simulink model "SMDFR_rom_MCDET_v2_2022b"  (R2022b)
settings: Solver=ode1be  StartTime=0.0  StopTime=1500  FixedStep=0.5  RelTol=1e-3
model workspace: external: MATLAB File simulation_core_dualfluid_FI3_sim_rom_extract_MCDET_v2.m (data not in the file)
values from neighbouring files (symbols this model uses):
  A_fw = [13.6 9 9 9 9 9 9 9 9 9 9 13.6]    [SA_DualFluid.mat]
  A_wc = [10.9 10.3 10.3 10.3 10.3 10.3 10.3 10.3 10.3 10.3 10.3 10.9]    [SA_DualFluid.mat]
  h_fw = [6546 4305.1 4305.1 4305.1 4305.1 4305.1 4305.1 4305.1 4305.1 4305.1 4305.1 7629.5]    [SA_DualFluid.mat]
  h_wc = [27405.4 13833.4 13833.4 13833.4 13833.4 13833.4 13833.4 13833.4 13833.4 13833.4 13833.4 32177.3]    [SA_DualFluid.mat]
  Ncomps = 5    [LJ_test_sampled_vel_ACS_2_loop_1180.mat]
undefined symbols (not defined in the file or in its folder): alfa_c, alfa_f, beta, beta_i, C_i0, c_pc, c_pf, c_pw, Ce_i0, complementary_branch_flag, DiscIntNeverNeededParam, failed_states, fault_time, initial_branch_state, initial_state, L, Lambda, lambda_c, lambda_e, lambda_i, M_c, M_f, M_w, mat_states_index, mat_trans, mdot_c, mdot_c_drift, mdot_f, N_0, Nstates, P_0, parent_last_time, Pi_0, rho_0, rhoex_value, Tbar_c0, Tbar_f0, Tc_0, Tf_0, Tin_f0, Tw_0, vel_ACS
libraries: dspsrcs4 x1
settings Model: Creator=leona  LastModifiedBy=leona
settings DataIOCC: LoadExternalInput=on
settings OptimizationCC: ReuseModelBlockBuffer=on

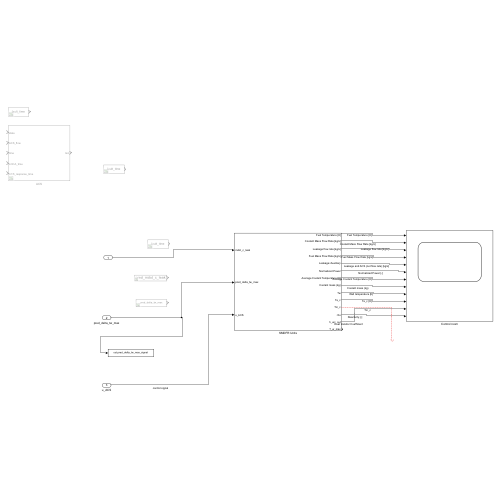
[thumbnail: Simulink's stored preview of the top-level diagram]
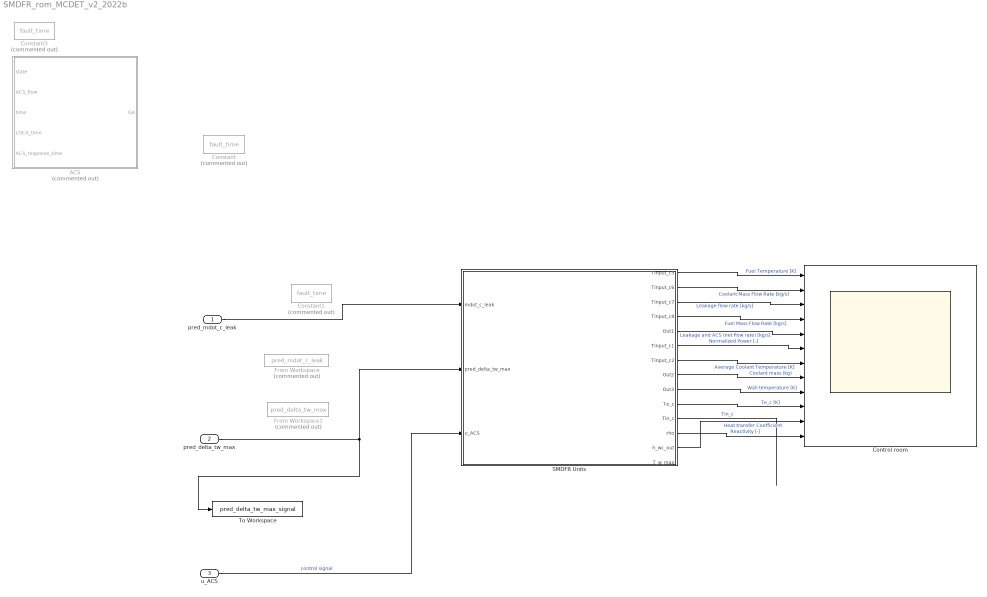
== system SMDFR_rom_MCDET_v2_2022b ==
  pred_mdot_c_leak : Inport
  pred_delta_tw_max : Inport  Port=2
  u_ACS : Inport  Port=3
  ACS : Subsystem  Commented=on
  Constant : Constant  Commented=on  Value=fault_time
  Constant1 : Constant  Commented=on  Value=fault_time
  Constant3 : Constant  Commented=on  Value=fault_time
  Control room : Scope  NumInputPorts=12
  From Workspace : FromWorkspace  Commented=on  VariableName=pred_mdot_c_leak  SampleTime=0.5  Interpolate=off  OutputAfterFinalValue=Holding final value
  From Workspace1 : FromWorkspace  Commented=on  VariableName=pred_delta_tw_max  SampleTime=0.5  OutputAfterFinalValue=Holding final value
  SMDFR Units : Subsystem
  To Workspace : ToWorkspace  VariableName=pred_delta_tw_max_signal  SaveFormat=Timeseries  SampleTime=-1
  wires:
  SMDFR Units/1(Tinput_c5) -> Control room/1  "Fuel Temperature [K]"
  SMDFR Units/2(Tinput_c6) -> Control room/2  "Coolant Mass Flow Rate [kg/s]"
  SMDFR Units/3(Tinput_c7) -> Control room/3  "Leakage flow rate [kg/s]"
  SMDFR Units/4(Tinput_c8) -> Control room/4  "Fuel Mass Flow Rate [kg/s]"
  SMDFR Units/5(Out1) -> Control room/5  "Leakage and ACS (net flow rate) [kg/s]"
  SMDFR Units/6(Tinput_c1) -> Control room/6  "Normalized Power [-]"
  SMDFR Units/7(Tinput_c2) -> Control room/7  "Average Coolant Temperature [K]"
  SMDFR Units/8(Out2) -> Control room/8  "Coolant mass (kg)"
  SMDFR Units/9(Out3) -> Control room/9  "Wall temperature [K]"
  SMDFR Units/10(Te_c) -> Control room/10  "Te_c [K]"
  SMDFR Units/11(Tin_c) -> ?  "Tin_c"
  SMDFR Units/12(rho) -> Control room/12  "Reactivity [-]"
  SMDFR Units/13(h_wc_out) -> Control room/11  "Heat transfer Coefficient"
  pred_delta_tw_max/1 -> To Workspace/1, SMDFR Units/2(pred_delta_tw_max)
  pred_mdot_c_leak/1 -> SMDFR Units/1(mdot_c_leak)
  u_ACS/1 -> SMDFR Units/3(u_ACS)  "control signal"

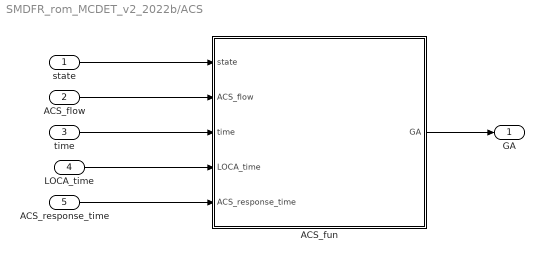
== system SMDFR_rom_MCDET_v2_2022b/ACS ==
  state : Inport
  ACS_flow : Inport  Port=2
  time : Inport  Port=3
  LOCA_time : Inport  Port=4
  ACS_response_time : Inport  Port=5
  ACS_fun : MATLAB Function  TreatAsAtomicUnit=on
  GA : Outport
  wires:
  ACS_flow/1 -> ACS_fun/2(ACS_flow)
  state/1 -> ACS_fun/1(state)
  ACS_fun/1(GA) -> GA/1
  time/1 -> ACS_fun/3(time)
  LOCA_time/1 -> ACS_fun/4(LOCA_time)
  ACS_response_time/1 -> ACS_fun/5(ACS_response_time)

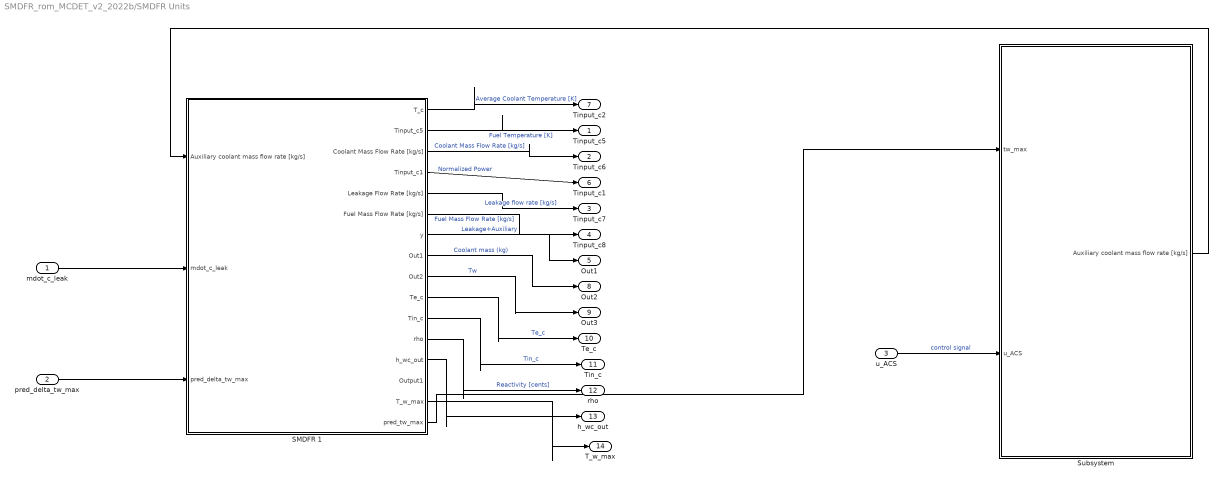
== system SMDFR_rom_MCDET_v2_2022b/SMDFR Units ==
  mdot_c_leak : Inport
  pred_delta_tw_max : Inport  Port=2
  u_ACS : Inport  Port=3
  SMDFR 1 : Subsystem
  Subsystem : Subsystem
  Tinput_c5 : Outport
  Tinput_c6 : Outport  Port=2
  Tinput_c7 : Outport  Port=3
  Tinput_c8 : Outport  Port=4
  Out1 : Outport  Port=5
  Tinput_c1 : Outport  Port=6
  Tinput_c2 : Outport  Port=7
  Out2 : Outport  Port=8
  Out3 : Outport  Port=9
  Te_c : Outport  Port=10
  Tin_c : Outport  Port=11
  rho : Outport  Port=12
  h_wc_out : Outport  Port=13
  T_w_max : Outport  Port=14
  wires:
  SMDFR 1/10(Te_c) -> Te_c/1  "Te_c"
  SMDFR 1/8(Out1) -> Out2/1  "Coolant mass (kg)"
  SMDFR 1/12(rho) -> rho/1  "Reactivity [cents]"
  SMDFR 1/9(Out2) -> Out3/1  "Tw"
  SMDFR 1/1(T_c) -> Tinput_c2/1  "Average Coolant Temperature [K]"
  SMDFR 1/3(Coolant Mass Flow Rate [kg/s]) -> Tinput_c6/1  "Coolant Mass Flow Rate [kg/s]"
  SMDFR 1/11(Tin_c) -> Tin_c/1  "Tin_c"
  SMDFR 1/6(Fuel Mass Flow Rate [kg/s]) -> Tinput_c8/1  "Fuel Mass Flow Rate [kg/s]"
  SMDFR 1/4(Tinput_c1) -> Tinput_c1/1  "Normalized Power"
  SMDFR 1/7(y) -> Out1/1  "Leakage+Auxiliary"
  SMDFR 1/2(Tinput_c5) -> Tinput_c5/1  "Fuel Temperature [K]"
  SMDFR 1/5(Leakage Flow Rate [kg/s]) -> Tinput_c7/1  "Leakage flow rate [kg/s]"
  Subsystem/1(Auxiliary coolant mass flow rate [kg/s]) -> SMDFR 1/1(Auxiliary coolant mass flow rate [kg/s])
  SMDFR 1/13(h_wc_out) -> h_wc_out/1
  SMDFR 1/15(T_w_max) -> T_w_max/1
  SMDFR 1/16(pred_tw_max) -> Subsystem/1(tw_max)
  mdot_c_leak/1 -> SMDFR 1/2(mdot_c_leak)
  pred_delta_tw_max/1 -> SMDFR 1/3(pred_delta_tw_max)
  u_ACS/1 -> Subsystem/2(u_ACS)  "control signal"

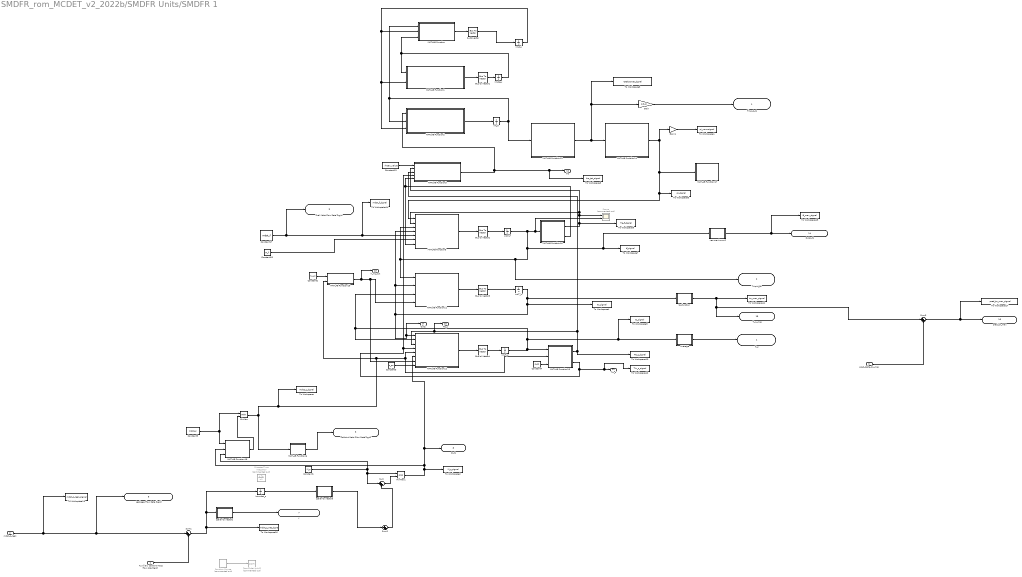
== system SMDFR_rom_MCDET_v2_2022b/SMDFR Units/SMDFR 1 ==
  Auxiliary coolant mass flow rate [kg/s] : Inport
  mdot_c_leak : Inport  Port=2
  pred_delta_tw_max : Inport  Port=3
  Average : MATLAB Function  TreatAsAtomicUnit=on
  Bus to Vector{1..4} (4 alike) : BusToVector
  Constant1 : Constant  Value=M_c
  Constant13 : Constant  Value=rhoex_value  SampleTime=-1
  Constant17 : Constant  Value=mdot_f  SampleTime=-1
  Constant2 : Constant  Value=h_wc
  Constant20 : Constant  Value=M_f  SampleTime=-1
  Constant3 : Constant  Value=c_pc
  Constant4 : Constant  Value=c_pc
  Constant9 : Constant  Value=mdot_c  SampleTime=-1
  Discrete-Time Integrator : DiscreteIntegrator  Commented=on  SampleTime=0.5  ICPrevOutput=DiscIntNeverNeededParam  ICPrevScaledInput=DiscIntNeverNeededParam
  Gain : Gain  Gain=1/P_0
  Gain1 : Gain  Gain=1/P_0
  Int-C_i : Integrator  InitialCondition=C_i0
  Int-Ce_i : Integrator  InitialCondition=Ce_i0
  Int-T_c : Integrator  InitialCondition=Tc_0
  Int-T_f : Integrator  InitialCondition=Tf_0
  Int-T_w : Integrator  InitialCondition=Tw_0
  Int-mdot_c : Integrator
  Int_N : Integrator  InitialCondition=N_0
  MATLAB Function : MATLAB Function  TreatAsAtomicUnit=on
  MATLAB Function1 : MATLAB Function  TreatAsAtomicUnit=on
  MATLAB Function11 : MATLAB Function  TreatAsAtomicUnit=on
  MATLAB Function12 : MATLAB Function  TreatAsAtomicUnit=on
  MATLAB Function13 : MATLAB Function  TreatAsAtomicUnit=on
  MATLAB Function14 : MATLAB Function  TreatAsAtomicUnit=on
  MATLAB Function15 : MATLAB Function  TreatAsAtomicUnit=on
  MATLAB Function16 : MATLAB Function  TreatAsAtomicUnit=on
  MATLAB Function17 : MATLAB Function  TreatAsAtomicUnit=on
  MATLAB Function18 : MATLAB Function  TreatAsAtomicUnit=on
  MATLAB Function19 : MATLAB Function  TreatAsAtomicUnit=on
  MATLAB Function2 : MATLAB Function  TreatAsAtomicUnit=on
  MATLAB Function3 : MATLAB Function  TreatAsAtomicUnit=on
  MATLAB Function5 : MATLAB Function  TreatAsAtomicUnit=on
  MATLAB Function6 : MATLAB Function  TreatAsAtomicUnit=on
  MinMax : MinMax  Inputs=2
  MinMax1 : MinMax  Inputs=2
  Random Source : dspsrcs4/Random Source  Commented=on  SrcType=Gaussian  NormMethod=Ziggurat  CltLength=12  MinVal=0  MaxVal=1  MeanVal=0  VarVal=0.05*mdot_c_drift  RepMode=Not repeatable  rawSeed=1  IsInherit=off  SampMode=Discrete  SampTime=-1  SampFrame=1  DataType=Double  OutComplex=Real  OutputFrames=off
  Scope : Scope  Commented=on  NumInputPorts=2
  Sum{,1..3} (4 alike) : Sum  Inputs=|++
  To Workspace : ToWorkspace  VariableName=mdot_c_signal  SaveFormat=Timeseries  SampleTime=-1
  To Workspace1 : ToWorkspace  VariableName=pi_normsignal  SaveFormat=Timeseries  SampleTime=-1
  To Workspace10 : ToWorkspace  VariableName=Te_c_signal  SaveFormat=Timeseries  SampleTime=-1
  To Workspace11 : ToWorkspace  VariableName=tw_max_signal  SaveFormat=Timeseries  SampleTime=-1
  To Workspace12 : ToWorkspace  VariableName=Tin_c_signal  SaveFormat=Timeseries  SampleTime=-1
  To Workspace13 : ToWorkspace  VariableName=mdot_c_leak_signal  SaveFormat=Timeseries  SampleTime=-1
  To Workspace14 : ToWorkspace  VariableName=mdot_f_signal  SaveFormat=Timeseries  SampleTime=-1
  To Workspace15 : ToWorkspace  VariableName=tf_max_signal  SaveFormat=Timeseries  SampleTime=-1
  To Workspace16 : ToWorkspace  VariableName=mdot_c_net_signal  SaveFormat=Timeseries  SampleTime=-1
  To Workspace17 : ToWorkspace  VariableName=pred_tw_max_signal  SaveFormat=Timeseries  SampleTime=-1
  To Workspace2 : ToWorkspace  VariableName=M_c_signal  SaveFormat=Timeseries  SampleTime=-1
  To Workspace3 : ToWorkspace  VariableName=totalpower_signal  SaveFormat=Timeseries  SampleTime=-1
  To Workspace4 : ToWorkspace  VariableName=tw_signal  SaveFormat=Timeseries  SampleTime=-1
  To Workspace5 : ToWorkspace  VariableName=tc_signal  SaveFormat=Timeseries  SampleTime=-1
  To Workspace6 : ToWorkspace  VariableName=pi_signal  SaveFormat=Timeseries  SampleTime=-1
  To Workspace7 : ToWorkspace  VariableName=tf_signal  SaveFormat=Timeseries  SampleTime=-1
  To Workspace8 : ToWorkspace  VariableName=rho_tot_signal  SaveFormat=Timeseries  SampleTime=-1
  To Workspace9 : ToWorkspace  VariableName=Te_f_signal  SaveFormat=Timeseries  SampleTime=-1
  Zero-Order Hold2 : ZeroOrderHold  Commented=on  SampleTime=-1
  bustovector : BusToVector
  scalar to vector2 : MATLAB Function  TreatAsAtomicUnit=on
  scalar to vector3 : MATLAB Function  TreatAsAtomicUnit=on
  tp_function : MATLAB Function  TreatAsAtomicUnit=on
  vec maximum2 : MATLAB Function  TreatAsAtomicUnit=on
  T_c : Outport
  Tinput_c5 : Outport  Port=2
  Coolant Mass Flow Rate [kg/s] : Outport  Port=3
  Tinput_c1 : Outport  Port=4
  Leakage Flow Rate [kg/s] : Outport  Port=5
  Fuel Mass Flow Rate [kg/s] : Outport  Port=6
  y : Outport  Port=7
  Out1 : Outport  Port=8
  Out2 : Outport  Port=9
  Te_c : Outport  Port=10
  Tin_c : Outport  Port=11
  rho : Outport  Port=12
  h_wc_out : Outport  Port=13
  Output1 : Outport  Port=14
  T_w_max : Outport  Port=15
  pred_tw_max : Outport  Port=16
  wires:
  Constant20/1 -> MATLAB Function5/6(M_f)
  bustovector/1 -> Int-C_i/1
  Constant13/1 -> MATLAB Function3/1(rho_ext)
  Int-T_w/1 -> To Workspace4/1, Out2/1, MATLAB Function12/1(T_w), MATLAB Function5/4(T_w), MATLAB Function11/2(T_w), tp_function/1(T_w)  "Tw"
  MinMax/1 -> To Workspace/1, MATLAB Function19/2(mdot_c), MATLAB Function15/2(mdot_c), MATLAB Function12/5(mdot_c), MATLAB Function6/1(u)  "Coolant mass flow rate (kg/s)"
  scalar to vector2/1(y) -> y/1  "Auxiliary+leakage"
  MATLAB Function15/1(Te_c) -> To Workspace10/1, MATLAB Function3/3(Te_c), MATLAB Function12/3(Te_c), Te_c/1  "Te_c"
  MATLAB Function16/1(Te_f) -> To Workspace9/1, Scope/1, MATLAB Function3/2(Te_f), MATLAB Function5/2(Te_f)
  Constant17/1 -> Fuel Mass Flow Rate [kg/s]/1, To Workspace14/1, MATLAB Function5/5(mdot_f)  "Fuel mass flow rate (kg/s)"
  Bus to Vector4/1 -> Int-T_c/1
  MATLAB Function11/1(dT_wdt) -> Bus to Vector3/1
  MATLAB Function/1(dC_idt) -> bustovector/1
  MATLAB Function3/1(rho) -> MATLAB Function2/1(rho), To Workspace8/1, rho/1  "Total Reactivity (cents)"
  Constant9/1 -> MATLAB Function18/1(mdot_c), MinMax/1
  Int-Ce_i/1 -> MATLAB Function/3(Ce_i), MATLAB Function1/1(Ce_i)
  MATLAB Function12/1(dT_cdt) -> Bus to Vector4/1
  MATLAB Function13/1(P) -> To Workspace3/1, Gain/1, MATLAB Function14/1(P)
  MATLAB Function14/1(Pi) -> To Workspace6/1, MATLAB Function5/1(Pi), MATLAB Function17/1(Pi), Gain1/1
  MATLAB Function5/1(dT_fdt) -> Bus to Vector2/1
  Bus to Vector2/1 -> Int-T_f/1
  Bus to Vector1/1 -> Int-Ce_i/1
  MATLAB Function1/1(dCei_dt) -> Bus to Vector1/1
  Int-C_i/1 -> MATLAB Function2/3(C_i), MATLAB Function1/2(C_i), MATLAB Function/2(C_i)
  MATLAB Function2/1(dN_dt) -> Int_N/1
  Int_N/1 -> MATLAB Function13/1(N), MATLAB Function/1(N), MATLAB Function2/2(N)
  Bus to Vector3/1 -> Int-T_w/1
  Average/1(y) -> T_c/1  "Average Coolant Temperature [K]"
  Int-T_c/1 -> MATLAB Function12/2(T_c), MATLAB Function11/3(T_c), To Workspace5/1, Average/1(u), MATLAB Function15/1(T_c)  "Coolant Temperature [K]"
  MATLAB Function6/1(y) -> Coolant Mass Flow Rate [kg/s]/1
  Auxiliary coolant mass flow rate [kg/s]/1 -> Sum1/2  "Auxiliary coolant mass flow rate [kg/s]"
  MATLAB Function18/1(y) -> MinMax/2  "Coolant mass flow rate (kg/s)"
  scalar to vector3/1(y) -> Sum2/1  "Coolant mass per node (kg)"
  Constant1/1 -> Sum/1, MinMax1/1, MATLAB Function18/3(M_total)
  MATLAB Function15/2(Tin_c) -> MATLAB Function3/4(Tin_c), MATLAB Function12/4(Tinput_c), To Workspace12/1, Tin_c/1  "Tin_c"
  MinMax1/1 -> To Workspace2/1, MATLAB Function12/6(M_c), Out1/1, MATLAB Function18/2(M_actual)  "Coolant mass (kg)"
  Constant2/1 -> MATLAB Function19/1(h_wc)
  MATLAB Function19/1(h_wc_out) -> h_wc_out/1, MATLAB Function12/7(h_wc), MATLAB Function11/4(h_wc)
  Sum/1 -> MinMax1/2  "Coolant mass (kg)"
  Random Source/1 -> Zero-Order Hold2/1
  Gain/1 -> Tinput_c1/1  "Normalized Power"
  Gain1/1 -> To Workspace1/1
  MATLAB Function16/2(Tin_f) -> MATLAB Function3/5(Tin_f), MATLAB Function5/7(Tin_f)
  Int-mdot_c/1 -> scalar to vector3/1(u)  "Coolant mass per node (kg)"
  Int-T_f/1 -> vec maximum2/1(T_f), To Workspace7/1, Tinput_c5/1, MATLAB Function11/1(T_f), MATLAB Function5/3(T_f), Scope/2, MATLAB Function16/1(T_f)  "Fuel temperature profile (K)"
  vec maximum2/1(y) -> To Workspace15/1, Output1/1  "T_f_max"
  Sum2/1 -> Sum/2
  Constant3/1 -> MATLAB Function12/8(c_pc)
  Constant4/1 -> MATLAB Function15/3(c_pc)
  Sum1/1 -> Int-mdot_c/1, scalar to vector2/1(u), To Workspace16/1
  mdot_c_leak/1 -> Sum1/1, Leakage Flow Rate [kg/s]/1, To Workspace13/1
  Sum3/1 -> To Workspace17/1, pred_tw_max/1
  pred_delta_tw_max/1 -> Sum3/2
  tp_function/1(T_p) -> Sum3/1, T_w_max/1, To Workspace11/1

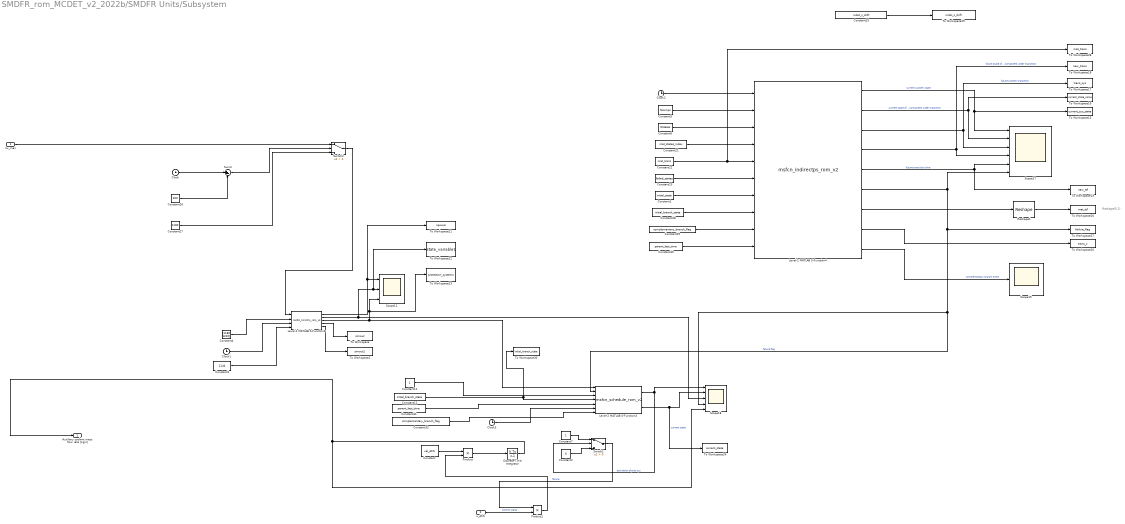
== system SMDFR_rom_MCDET_v2_2022b/SMDFR Units/Subsystem ==
  note: Reshape(5,2)
  tw_max : Inport
  u_ACS : Inport  Port=2
  Clock{,1..3} (4 alike) : Clock
  Constant : Constant  Value=vel_ACS
  Constant1 : Constant  Value=initial_state
  Constant11 : Constant  Value=initial_branch_state
  Constant12 : Constant
  Constant2 : Constant  Value=0
  Constant21 : Constant  Value=mat_states_index
  Constant22 : Constant  Value=mat_trans
  Constant23 : Constant  Value=failed_states
  Constant25 : Constant  Value=mdot_c_drift
  Constant26 : Constant  Value=200
  Constant27 : Constant  Value=1100
  Constant28 : Constant  Value=initial_branch_state
  Constant29 : Constant  Value=complementary_branch_flag
  Constant3 : Constant  Value=1144
  Constant30 : Constant  Value=parent_last_time
  Constant31 : Constant  Value=parent_last_time
  Constant32 : Constant  Value=complementary_branch_flag
  Constant4 : Constant  Value=[1180 1220]
  Constant5 : Constant  Value=Ncomps
  Constant6 : Constant  Value=Nstates
  Constant7 : Constant
  Discrete-Time Integrator : DiscreteIntegrator  SampleTime=-1  ICPrevOutput=DiscIntNeverNeededParam  ICPrevScaledInput=DiscIntNeverNeededParam
  Level-2 MATLAB S-Function2 : M-S-Function  FunctionName=msfcn_limintm_rom_v2
  Level-2 MATLAB S-Function3 : M-S-Function  FunctionName=msfcn_schedule_rom_v2
  Level-2 MATLAB S-Function4 : M-S-Function  FunctionName=msfcn_indirectps_rom_v2
  Product : Product
  Product1 : Product
  Reshape1 : Reshape  OutputDimensionality=Customize  OutputDimensions=[5,2]
  Scope11 : Scope  NumInputPorts=3
  Scope15 : Scope
  Scope17 : Scope  NumInputPorts=6
  Scope18 : Scope  NumInputPorts=5
  Sum3 : Sum  Inputs=|+-
  Switch1 : Switch  Criteria=u2 > Threshold  SaturateOnIntegerOverflow=off  InputSameDT=off
  Switch2 : Switch  Criteria=u2 > Threshold  SaturateOnIntegerOverflow=off  InputSameDT=off
  To Workspace : ToWorkspace  VariableName=simout  SaveFormat=Timeseries  SampleTime=-1
  To Workspace1 : ToWorkspace  VariableName=simout1  SaveFormat=Timeseries  SampleTime=-1
  To Workspace15 : ToWorkspace  VariableName=current_sys_state  SaveFormat=Timeseries  SampleTime=-1
  To Workspace16 : ToWorkspace  VariableName=current_state_comp  SaveFormat=Timeseries  SampleTime=-1
  To Workspace17 : ToWorkspace  VariableName=trans_sys  SaveFormat=Timeseries  SampleTime=-1
  To Workspace18 : ToWorkspace  VariableName=new_trans  SaveFormat=Timeseries  SampleTime=-1
  To Workspace19 : ToWorkspace  VariableName=new_ttf  SaveFormat=Timeseries  SampleTime=-1
  To Workspace20 : ToWorkspace  VariableName=trans_c  SaveFormat=Timeseries  SampleTime=-1
  To Workspace21 : ToWorkspace  VariableName=npower  SaveFormat=Timeseries  SampleTime=-1
  To Workspace22 : ToWorkspace  VariableName=state_variable1  SaveFormat=Timeseries  SampleTime=-1
  To Workspace23 : ToWorkspace  VariableName=protection_systems  SaveFormat=Timeseries  SampleTime=-1
  To Workspace24 : ToWorkspace  VariableName=current_state  SaveFormat=Timeseries  SampleTime=-1
  To Workspace26 : ToWorkspace  VariableName=mat_ttf  SaveFormat=Timeseries  SampleTime=-1
  To Workspace27 : ToWorkspace  VariableName=failure_flag  SaveFormat=Timeseries  SampleTime=-1
  To Workspace28 : ToWorkspace  VariableName=mat_trans  SaveFormat=Timeseries  SampleTime=-1
  To Workspace29 : ToWorkspace  VariableName=mdot_c_drift  SaveFormat=Timeseries  SampleTime=-1
  To Workspace30 : ToWorkspace  VariableName=initial_branch_state  SaveFormat=Timeseries  SampleTime=-1
  Auxiliary coolant mass flow rate [kg/s] : Outport
  wires:
  Level-2 MATLAB S-Function4/6 -> Level-2 MATLAB S-Function3/2, Scope18/4, To Workspace27/1, Scope17/6  "failure flag"
  Constant6/1 -> Level-2 MATLAB S-Function4/3
  Level-2 MATLAB S-Function4/9 -> Scope15/1  "complementary branch event"
  Sum3/1 -> Switch2/2
  Level-2 MATLAB S-Function4/5 -> To Workspace19/1, Scope17/5  "future transition time"
  Constant23/1 -> Level-2 MATLAB S-Function4/6
  Constant28/1 -> Level-2 MATLAB S-Function4/8
  Clock2/1 -> Level-2 MATLAB S-Function4/1
  Level-2 MATLAB S-Function2/2 -> Scope18/3, To Workspace22/1, Scope11/2
  Constant22/1 -> To Workspace28/1, Level-2 MATLAB S-Function4/5
  Discrete-Time Integrator/1 -> Auxiliary coolant mass flow rate [kg/s]/1, Scope18/5
  Level-2 MATLAB S-Function3/2 -> To Workspace24/1, Scope18/2  "current state"
  Level-2 MATLAB S-Function4/1 -> Scope17/1, To Workspace15/1  "current system state"
  Level-2 MATLAB S-Function4/4 -> Scope17/4, To Workspace18/1  "future state of component under transition"
  Clock3/1 -> Level-2 MATLAB S-Function3/6
  Constant21/1 -> Level-2 MATLAB S-Function4/4
  Constant32/1 -> Level-2 MATLAB S-Function3/7
  Level-2 MATLAB S-Function2/3 -> To Workspace23/1, Scope11/3, Level-2 MATLAB S-Function3/1
  Constant11/1 -> To Workspace30/1, Level-2 MATLAB S-Function3/4
  Constant30/1 -> Level-2 MATLAB S-Function4/10
  Constant31/1 -> Level-2 MATLAB S-Function3/5
  Reshape1/1 -> To Workspace26/1
  Constant12/1 -> Level-2 MATLAB S-Function3/3
  Level-2 MATLAB S-Function4/3 -> Scope17/3, To Workspace17/1  "future system transition"
  Clock/1 -> Sum3/1
  Clock1/1 -> Level-2 MATLAB S-Function2/3
  Constant1/1 -> Level-2 MATLAB S-Function4/7
  Level-2 MATLAB S-Function4/2 -> Scope17/2, To Workspace16/1  "current state of component under transition"
  Constant3/1 -> Level-2 MATLAB S-Function2/4
  Constant4/1 -> Level-2 MATLAB S-Function2/2
  Level-2 MATLAB S-Function4/7 -> Reshape1/1
  Constant7/1 -> Switch1/1
  Constant2/1 -> Switch1/3
  Level-2 MATLAB S-Function2/1 -> To Workspace21/1, Scope11/1
  Switch2/1 -> Level-2 MATLAB S-Function2/1
  Constant27/1 -> Switch2/3
  Constant26/1 -> Sum3/2
  Constant29/1 -> Level-2 MATLAB S-Function4/9
  Level-2 MATLAB S-Function3/1 -> Switch1/2, Scope18/1  "activation of prot sys"
  Constant5/1 -> Level-2 MATLAB S-Function4/2
  Level-2 MATLAB S-Function4/8 -> To Workspace20/1
  Constant25/1 -> To Workspace29/1
  tw_max/1 -> Switch2/1
  Level-2 MATLAB S-Function2/4 -> To Workspace/1
  Level-2 MATLAB S-Function2/5 -> To Workspace1/1
  Switch1/1 -> Product1/1  "failure"
  Constant/1 -> Product/1
  Product/1 -> Discrete-Time Integrator/1
  u_ACS/1 -> Product1/2  "control signal"
  Product1/1 -> Product/2

== matlab function SMDFR_rom_MCDET_v2_2022b/SMDFR Units/SMDFR 1/tp_function ==
  data: T_w input size=1; T_p output
function T_p = fcn(T_w)

T_p = max(T_w);

== matlab function SMDFR_rom_MCDET_v2_2022b/SMDFR Units/SMDFR 1/MATLAB Function11 ==
  data: T_f input size=1; T_w input size=1; dT_wdt output size=1; T_c input size=1; A_wc parameter size=1; A_fw parameter size=1; M_w parameter size=1; c_pw parameter size=1; h_wc input size=1; h_fw parameter size=1
function dT_wdt = eqn9(T_f, T_w, T_c, A_wc, A_fw, M_w, c_pw, h_wc, h_fw)
%dT_wdt = 0;

dT_wdt = ( h_fw*A_fw*(T_f - T_w) - h_wc*A_wc*(T_w -T_c) ) / (M_w * c_pw);

== matlab function SMDFR_rom_MCDET_v2_2022b/SMDFR Units/SMDFR 1/MATLAB Function12 ==
  data: T_w input size=1; T_c input size=1; A_wc parameter size=1; dT_cdt output size=1; Te_c input size=1; Tinput_c input; mdot_c input size=1; M_c input size=1; h_wc input size=1; c_pc input size=1
function dT_cdt = eqn10(T_w, T_c, A_wc, Te_c, Tinput_c, mdot_c, M_c, h_wc, c_pc)
%!!!
dT_cdt = 0;
%Tinput_c=Tinput_c(1);

dT_cdt = ( mdot_c*c_pc*(Tinput_c - Te_c) + h_wc*A_wc*(T_w - T_c) ) / (M_c * c_pc);

== matlab function SMDFR_rom_MCDET_v2_2022b/SMDFR Units/SMDFR 1/MATLAB Function13 ==
  data: P output; N input; N_0 parameter; P_0 parameter
function P = eqn14(N, N_0, P_0)
%P = P_0;

P = (P_0/N_0) * N;

== matlab function SMDFR_rom_MCDET_v2_2022b/SMDFR Units/SMDFR 1/MATLAB Function14 ==
  data: Pi output size=1; P input; Pi_0 parameter size=1; P_0 parameter
function Pi = distr(P, Pi_0, P_0)
Pi = 0;
%Pi = P_0*Pi_0';

Pi = P*Pi_0;

== matlab function SMDFR_rom_MCDET_v2_2022b/SMDFR Units/SMDFR 1/MATLAB Function15 ==
  data: T_c input size=1; Te_c output size=1; Te_c0 parameter size=1; mdot_c input size=1; Tin_c output size=1; c_pc input size=1
function [Te_c, Tin_c]  = cons1(T_c, Te_c0, mdot_c, c_pc)
%Te_c = tc_last;
%!!!
Te_c = Te_c0;

Q0 = 8.2564e+07*0.578;
Q = Q0*mdot_c(1)/(5550/2)-(5500-mdot_c);
Tin_c = Te_c-Q/(mean(mdot_c)*c_pc);

Te_c = 2*T_c - Tin_c;

== matlab function SMDFR_rom_MCDET_v2_2022b/SMDFR Units/SMDFR 1/MATLAB Function16 ==
  data: T_f input size=1; Te_f output size=1; Te_f0 parameter size=1; Tin_f output size=1
 function [Te_f, Tin_f] = cons1(T_f,Te_f0)
%Te_f = tf_last;
%Te_f = zeros(3,1);
%Te_f(2) = Te_f0(2);
%Te_f(3) = Te_f0(3);
%!!!
Te_f = Te_f0;
Tin_f = Te_f;
%Te_f(1) = Te_f0(1);

Te_f = 2*T_f - Tin_f;

== matlab function SMDFR_rom_MCDET_v2_2022b/SMDFR Units/SMDFR 1/MATLAB Function17 ==
  data: Pi input size=1; sum_P output
function sum_P = fcn(Pi)

sum_P = sum(Pi);

== matlab function SMDFR_rom_MCDET_v2_2022b/SMDFR Units/SMDFR 1/MATLAB Function18 ==
  data: mdot_c input; y output; M_actual input; M_total input
function y = fcn(mdot_c,M_actual,M_total)
y=0;

%y = mdot_c+Auxiliary_leakage*(time-LOCA_time);
y = mdot_c*M_actual/M_total;

== matlab function SMDFR_rom_MCDET_v2_2022b/SMDFR Units/SMDFR 1/vec maximum2 ==
  data: T_f input; y output
function y = fcn(T_f)

y = max(T_f);

== matlab function SMDFR_rom_MCDET_v2_2022b/SMDFR Units/SMDFR 1/MATLAB Function19 ==
  data: h_wc input; h_wc_out output; mdot_c input
function h_wc_out = fcn(h_wc,mdot_c)

h_wc_out=0;

h_wc_out=h_wc*(mdot_c/5550)^(0.8);

== matlab function SMDFR_rom_MCDET_v2_2022b/SMDFR Units/SMDFR 1/scalar to vector2 ==
  data: u input; y output
function y = fcn(u)
%!!!
y = 0;

y = u;

== matlab function SMDFR_rom_MCDET_v2_2022b/SMDFR Units/SMDFR 1/MATLAB Function6 ==
  data: u input; y output
function y = fcn(u)

y = mean(u);

== matlab function SMDFR_rom_MCDET_v2_2022b/SMDFR Units/SMDFR 1/MATLAB Function1 ==
  data: Ce_i input size=6,1; dCei_dt output size=6,1; C_i input size=6,1; lambda_i parameter size=1,6; lambda_e parameter; lambda_c parameter; L parameter
function dCei_dt = eqn3(Ce_i, C_i, lambda_i, lambda_e, lambda_c, L)
dCei_dt = zeros(6,1); %!!!

for i=1:L 
    dCei_dt(i) = -lambda_i(i)*Ce_i(i) - lambda_e*Ce_i(i) + lambda_c*C_i(i) ;
end

== matlab function SMDFR_rom_MCDET_v2_2022b/ACS/ACS_fun ==
  data: state input; GA output; ACS_flow input; time input; LOCA_time input; ACS_response_time input
function GA  = ACS(state,ACS_flow,time,LOCA_time,ACS_response_time)

if state && (time-LOCA_time) > ACS_response_time
    GA = ACS_flow;
else
    GA = 0;
end

== matlab function SMDFR_rom_MCDET_v2_2022b/SMDFR Units/SMDFR 1/MATLAB Function ==
  data: N input; dC_idt output size=6,1; C_i input size=6,1; Ce_i input size=6,1; Lambda parameter; lambda_i parameter size=1,6; lambda_c parameter; lambda_e parameter; beta_i parameter size=1,6
function dC_idt = eqn2(N, C_i, Ce_i, Lambda, lambda_i, lambda_c, lambda_e, beta_i)
dC_idt = zeros(6,1);

for i=1:6
    dC_idt(i) = beta_i(i)/Lambda * N - lambda_i(i)*C_i(i) - lambda_c*C_i(i) + lambda_e*Ce_i(i);
end

== matlab function SMDFR_rom_MCDET_v2_2022b/SMDFR Units/SMDFR 1/MATLAB Function2 ==
  data: rho input; dN_dt output; N input; C_i input size=6,1; lambda_i parameter size=1,6; beta parameter; Lambda parameter; L parameter
function dN_dt = eqn4(rho, N, C_i, lambda_i, beta, Lambda, L)
sum_i = 0;

for i=1:L 
    sum_i = sum_i + lambda_i(i)*C_i(i);
end

dN_dt = (rho - beta)*(N/Lambda) + sum_i;

== matlab function SMDFR_rom_MCDET_v2_2022b/SMDFR Units/SMDFR 1/MATLAB Function3 ==
  data: rho_ext input; rho output; rho_0 parameter; Te_f input; Te_c input; Tbar_f0 parameter; Tbar_c0 parameter; alfa_f parameter; alfa_c parameter; Tin_c input; Tin_f input; Tin_f0 parameter
function rho = eqn15(rho_ext, rho_0, Te_f, Te_c, Tbar_f0, Tbar_c0, alfa_f, alfa_c, Tin_c, Tin_f, Tin_f0)

rho = rho_0 + alfa_f*(mean([Te_f,Tin_f]) - Tbar_f0) + alfa_c*(mean([Te_c,Tin_c]) - Tbar_c0) + rho_ext;

== matlab function SMDFR_rom_MCDET_v2_2022b/SMDFR Units/SMDFR 1/Average ==
  data: u input; y output
function y = fcn(u)

y = mean(u);

== matlab function SMDFR_rom_MCDET_v2_2022b/SMDFR Units/SMDFR 1/scalar to vector3 ==
  data: u input; y output size=1; M_c parameter
function y = fcn(u, M_c)
%!!!
y = 0;
%for i = 1:3
    %if i == 2
y = u*(M_c/sum(M_c));
    %else
       % y(i) = u*0.027;
    %end
%end

== matlab function SMDFR_rom_MCDET_v2_2022b/SMDFR Units/SMDFR 1/MATLAB Function5 ==
  data: Pi input size=1; dT_fdt output size=1; Te_f input size=1; T_f input size=1; T_w input size=1; c_pf parameter size=1; h_fw parameter size=1; A_fw parameter size=1; mdot_f input size=1; M_f input size=1; Tin_f input; Tin_f0 parameter
function dT_fdt = eqn8(Pi, Te_f, T_f, T_w, c_pf, h_fw, A_fw, mdot_f, M_f, Tin_f, Tin_f0)
dT_fdt=0;

dT_fdt = ( Pi + mdot_f * c_pf * (Tin_f - Te_f) - h_fw*A_fw*(T_f - T_w) ) / (M_f * c_pf);
